simulink library "PacketizedNetworkLib"  (R2025b)
settings: Solver=VariableStepAuto  StartTime=0.0  StopTime=10.0  RelTol=1e-3
values from neighbouring files (symbols this model uses):
  dfeRef = [0.707106781187 -0.707106781187 0.707106781187 0.707106781187 -0.707106781187 0.707106781187 0.707106781187 0.707106781187 0.707106781187 0.707106781187 -0.707106781187 0.707106781187 ... (500 elements, 500x1)]    [networkParams.mat]
  L3payload = [0 0 0 1 0 0 0 0 1 1 1 0 ... (1040 elements, 1040x1)]    [networkParams.mat]
  ppdu_bb = [0 0 1 1 0 0 0 0 1 1 0 0 ... (2280 elements, 2280x1)]    [networkParams.mat]
  Ts = 1e-07    [networkParams.mat]
undefined symbols (not defined in the file or in its folder): AckDestAddre, DestAddre, dfilt, High, lambda, NodeAddre, pseed
libraries: $bdroot x19, hdlsllib x5, dspsigops x5, dspswit3 x3, simulink x3, dspindex x3, commdigbbndpm3 x2, simulink_extras x2, commfilt2 x2, commchan3 x1, dspmathops x1, dsparch4 x1
(part 3 of 3)

== stateflow chart PacketizedNetworkLib/PHY//MAC Transceiver/Subsystem/CSMA//CA MAC Layer ==
  note: Note:  802.11-like MAC with basic functions for DCF scenarios. PCF, HCF, MCF not implementaed.  For DCF, RTS and CTS  not implemented.
      |
      | 	    The MAC time unit is 8 times the symbol time (Ts), or 16 times the bit time.
      |           TxLength: data packet bit length divided by 16 = 529*(8000+464)/16.
      |   	    SLOT: backoff duration = TxLength/2.  With carrier sense or NAV, SLOT can be much smaller.
      |           CW: contention window length (number of SLOTs).
      | 	    BOTime: random back off time = randi([0 CW],1)*SLOT;
      |           AckLength: ack duration in MAC time units (number of ACK bits / 16)
      |           AckWaitTime: timer for AckWait state
      |           Retry is the retry number of a frame.
      |
      |           IFS Interfame space
      |           SigD Signal detection signal (i.e., carrier-sensing result)
      |           TxLength is an input from Link layer to indicate the bit length of the data packet.
      |           AckOK is the status of ACK packet CRC OK.
      |           TxDataTP is the time pading for the node to meet the SIFS time.
      |           TxAckTP is the time pading for the node to meet the SIFS time.
      |           TxDataDone is an output to LLC layer to show the current frame is transmitted OK.
      |           TxDataFail is an output to LLC layer to indicate that the current packet is failed.
  state Tx1 DATA and wait for ACK [group]
    state Reset
    state Reset1
    state TxOn
      en:
      TxTime=TxTime-1;
      TxDataOn=1;
    state AckWait
      en:
      AckWaitTime=AckWaitTime-1;
    state TurnOnTxSw
      en:
      TxDataTP=TxDataTP-1;
    Reset -> (junction 461) : {TxDataFail=0;}
    (junction 461) -> (junction 374)
    (junction 330) -> (junction 461) [order 1] : [Retry<SSCR]
        | {Retry=Retry+1;}
    (junction 327) -> (junction 374) [order 2] : {TxDataDone=0;}
    (junction 330) -> Reset [order 2] : [Retry==SSCR]
        | {TxDataFail=1;
        | Retry=0;
        | CW=CWmin; }
    Reset1 -> (junction 327)
    AckWait -> Reset1 [order 1] : [AckOk==1&&AckWaitTime>0]
        | {TxDataDone=1;
        | Retry=0;
        | CW=CWmin;}
    (junction 327) -> TurnOnTxSw [order 1] : [TxEn==1]
        | {BONum=0;
        | TxDataDone=0;
        | TxTime=TxLength;
        | TxDataTP=TP;}
    TxOn -> TxOn [order 2] : [TxTime>0]
    AckWait -> (junction 330) [order 2] : [AckWaitTime==0]
    TxOn -> AckWait [order 1] : [TxTime==0]
        | {AckWaitTime=AckLength+SIFS+20;
        | TxDataOn=0;}
    TurnOnTxSw -> TxOn [order 1] : [TxDataTP<=0]
    AckWait -> AckWait [order 3] : [AckWaitTime>0]
    TurnOnTxSw -> TurnOnTxSw [order 2]
  state Contention Window and Back Off [group]
    state IFS_Time
    state Backoff
      en:
      BOTime=BOTime-1;
    Backoff -> (junction 486) [order 1] : [SigD==1]
    IFS_Time -> IFS_Time [order 3] : [SigD==0]
        | {IFS=IFS-1;
        | SigSt=1;}
    IFS_Time -> (junction 473) [order 1] : [IFS==0]
    (junction 473) -> (junction 484) [order 2]
    (junction 484) -> (junction 354) [order 2]
    (junction 354) -> (junction 482) [order 2]
    (junction 473) -> Backoff [order 1] : [BOTime>0]
    (junction 484) -> Backoff [order 1] : [CW==CWmax]
        | {BOTime=randi([0 CW],1)*SLOT;}
    (junction 354) -> Backoff [order 1] : [Retry==0]
        | {BOTime=randi([0 CW],1)*SLOT;}
    (junction 482) -> Backoff : [CW<CWmax]
        | {CW=CW*2+1;
        | BOTime=randi([0 CW],1)*SLOT; }
    IFS_Time -> IFS_Time [order 5] : [RxErr==1]
        | {IFS=EIFS;}
    Backoff -> Backoff [order 3] : [BOTime>0&&SigD==0]
  state Tx ACK [group]
    state StandBy
    state RxDataOK
      en:
      TxAckTP=TxAckTP-1;
    state AckOn
      en:
      TxAckTime=TxAckTime-1;
      TxAckOn=1;
    (junction 434) -> StandBy [order 2]
    AckOn -> (junction 434) [order 1] : [TxAckTime==0]
        | {TxAckOn=0;
        | TxK=2;}
    StandBy -> (junction 394) [order 1] : [RxDataOk==1]
    (junction 394) -> RxDataOK : {TxAckTP=TP;}
    RxDataOK -> AckOn [order 1] : [TxAckTP<=0]
        | {TxAckTime=AckLength;}
    RxDataOK -> RxDataOK [order 2]
    AckOn -> AckOn [order 2]
  (default) -> (junction 372) : {
      | % Symbol time Ts = 1e-7, Bit time = Ts/2 = 0.5e-7.  MAC Clock Time is 16*(Ts/2) = 0.8 us
      | AckLength=400/16;      %Ack length = 400 bits, here "16" is the number of bits for MAC step size in bits
      | SLOT= 25;    %SLOT Time 20 us, 25*16*(Ts/2)= 20 us
      | DIFS = 62;    %DIFS Time  50 us, 62*16*(Ts/2)= 49.6 us
      | SIFS = 12;    %SIFS Time  10 us, 12*16*(Ts/2)= 9.6 us
      | EIFS = 100;  %EIFS Time  Ack Length + SIFS + DIFS, 20us + 50us + 10us = 80 us, 100*16*(Ts/2) = 80 us
      | TP=2;            % Tx/Rx Turnaround Time Padding for the node to meet SIFS time
      | rng(pseed) ;  % Rand Seed
      | CWmax=31;
      | CWmin=7;
      | TxDataFail=0;
      | TxDataDone=0;
      | BONum=0;
      | SSCR=10;
      | Retry=0;
      | %SigD=0;       % Signal detection is set to zero for the case that the carrier sense is not used in ALOHA MAC
      | }
  (junction 466) -> (junction 372) [order 2]
  (junction 374) -> (junction 466)
  (junction 372) -> StandBy : {CW=CWmin;
      | BONum=0;
      | BOTime=0;}
  (junction 466) -> (junction 488) [order 1] : [TxEn==1]
  (junction 486) -> (junction 488)
  (junction 488) -> (junction 452)
  (junction 434) -> (junction 452) [order 1] : [BOTime>0]
  StandBy -> (junction 452) [order 2] : [TxEn==1]
  (junction 452) -> IFS_Time : {IFS=DIFS;
      | SigSt=0;}
  IFS_Time -> (junction 452) [order 4] : [SigD==1&&SigSt==1]
  IFS_Time -> (junction 394) [order 2] : [RxDataOk==1]
  Backoff -> (junction 394) [order 2] : [RxDataOk==1]
  Backoff -> TurnOnTxSw [order 4] : [BOTime<=0]
      | {TxTime=TxLength;
      | TxDataTP=TP;}
  data: TxLength input double; TxEn input; RxDataOk input; AckOk input; TxDataFail output double; TxDataDone output double; AckLength local double; BONum local double; SIFS local double; CWmax local double; CW local double; SLOT local double; TxTime local double; TxDataOn output double; TxK local; TxAckOn output; BOTime output double; AckWaitTime output double; TxAckTP local; TxDataTP local; TP local; DIFS local; EIFS local; TxAckTime local; SigD input; SigSt local; RxErr input; IFS local; SSCR local; CWmin local; pseed parameter; Retry output

== matlab function PacketizedNetworkLib/PHY//MAC Transceiver/MATLAB Function ==
  data: ack output; NodeAddre parameter; DestAddre parameter; ppdu_bb parameter; AckDestAddre parameter
function ack = ackGenerator(NodeAddre, DestAddre, ppdu_bb, AckDestAddre)

%   Copyright 2017 The MathWorks, Inc.

persistent agc sync ackLength headCRC crcGenPHY crcGenMAC type version ...
            reserved sequenceNo fromAddress toAddress ackBits ackCRC 

% PHY Header

if isempty(crcGenMAC)
  agc  = ppdu_bb(1:50,1); %Load AGC signal
  sync = ppdu_bb(51:304); %Load Sync Signal
  ackLength = de2bi(64, 16, 'left-msb')';
  
  crcGenPHY = comm.CRCGenerator();
  temp = crcGenPHY(ackLength);
  headCRC = temp(17:32);
    
  % MAC header
  crcGenMAC = comm.CRCGenerator('z^32+z^26+z^23+z^22+z^16+z^12+z^11+z^10+z^8+z^7+z^5+z^4+z^2+z^1+1');
  type = [1 1 0 0]'; % [0 0 1 1] For Data Frame, [ 1 1 0 0] For ACK frame
  version = [0 0]';
  reserved = [0 0]';
  sequenceNo = [ 0 0 0 0 0 0 0 0 ]';
  
  toAddress = AckDestAddre';
  fromAddress = NodeAddre';

  ackBits=[type; ...
           version; ...
           reserved; ...
           toAddress; ...
           fromAddress; ...
           sequenceNo];

  ackCRC = crcGenMAC(ackBits);
end

ack =  [agc; ...
        sync; ...
        ackLength; ...
        headCRC; ...
        ackBits; ...
        ackCRC(end-31:end)];

== matlab function PacketizedNetworkLib/PHY//MAC Transceiver/MATLAB Function1 ==
  data: L3payload input size=1040; dataFrame output size=1472; NodeAddre parameter; DestAddre parameter; ppdu_bb parameter
function dataFrame = dataFrameGenerator(L3payload, NodeAddre, DestAddre, ppdu_bb)

%   Copyright 2017 The MathWorks, Inc.

persistent agc sync dataLength headCRC crcGenPHY crcGenMAC type version ...
            reserved sequenceNo fromAddress toAddress dataBits dataCRC ...
            time payload
          

% PHY Header

if isempty(crcGenMAC)
  agc  = ppdu_bb(1:50,1); %Load AGC signal
  sync = ppdu_bb(51:304); %Load Sync Signal
  dataLength = de2bi(64+length(L3payload)+32, 16, 'left-msb')';
  
  crcGenPHY = comm.CRCGenerator();
  temp = crcGenPHY(dataLength);
  headCRC = temp(17:32);
    
  % MAC header
  crcGenMAC = comm.CRCGenerator('z^32+z^26+z^23+z^22+z^16+z^12+z^11+z^10+z^8+z^7+z^5+z^4+z^2+z^1+1');
  type = [0 0 1 1]'; % [0 0 1 1] For Data Frame, [ 1 1 0 0] For ACK frame
  version = [0 0]';
  reserved = [0 0]';
  sequenceNo = [ 0 0 0 0 0 0 0 0 ]';
  time = zeros(32,1);
  
  fromAddress = NodeAddre';
  toAddress = DestAddre';

  payload = L3payload;
  
  dataBits=[type; ...
           version; ...
           reserved; ...
           toAddress; ...
           fromAddress; ...
           sequenceNo; ...
           time; ...
           payload];

  dataCRC = crcGenMAC(dataBits);
end

dataFrame =  [agc; ...
              sync; ...
              dataLength; ...
              headCRC; ...
              dataBits; ...
              dataCRC(end-31:end)];

== stateflow chart PacketizedNetworkLib/Logical Link Control/Logical Link Control ==
  state TxBackOn
    en:
    TxWaitTime=TxWaitTime-1;
    TxEn=0;
  state TxFailCount
    en:
    TxFlCnt=TxFlCnt+1 ;
  state TxPacket
    en:
    TxEn=1;
  note: Notes:
      |             TxWaitTime is the packet inter-arrival time. It represents multiples of 8*Ts.
      |             TxMore is a random number in [1 4], indicating additional segments transmissions.
      |             TxDataDone is an input from the MAC layer indicating that the current frame completed transmission.
      |             TxDataFail is an input from the MAC layer indicating that the current packet failed transmission.
      | 		TxDataBitsLength is the bit length of the data payload from layer #3 (network).
      |             TxLength is the frame length in multiples of 16 bits.
      |             StopSim is an output of the LLC that stops simulation when a frame completely fails transmission.
  (default) -> (junction 5) : {TxDataBitsLength=1040;  % M (Link payload)
      | TxFlCntMax=100;
      | TxLength=(TxDataBitsLength+464)/16; % 464 is the bit # of AGC+Header+MAC_Header+FCS
      | rng(pseed) ; % Poisson Rand Seed
      | TxFlCnt=0;
      | }
  TxFailCount -> (junction 5) [order 2] : [TxFlCnt<TxFlCntMax]
  TxFailCount -> (junction 10) [order 1] : [TxFlCnt==TxFlCntMax]
      | {StopSim=1;
      | TxEn=0;}
  (junction 5) -> TxBackOn : {
      | TxWaitTime=TxWaitUnits;
      | TxMore=randi([1 4], 1)-1;
      |  }
  TxPacket -> (junction 5) [order 1] : [TxDataDone==1&&TxMore<=0]
  TxBackOn -> TxBackOn [order 2]
  TxPacket -> TxFailCount [order 2] : [TxDataFail==1]
      | {TxEn=0;}
  TxBackOn -> TxPacket [order 1] : [TxWaitTime<=0]
  TxPacket -> TxPacket [order 3] : [TxDataDone==1]
      | {TxMore=TxMore-1;}
  data: TxDataDone input; TxDataFail input; StopSim output; TxEn output; TxDataBitsLength local; TxFlCnt local; TxFlCntMax local double; TxLength output; TxWaitTime output; TxMore output; pseed parameter; TxWaitUnits input

== matlab function PacketizedNetworkLib/Receiver/DFE /Sign_C  ==
  data: u input; y output
function y = fcn(u)
y=0.707*complex(sign(real(u)), sign(imag(u)));

== stateflow chart PacketizedNetworkLib/ALOHA MAC Layer ==
  state Delay
  state Reset
  state Tx1 DATA [group]
    state Reset1
    state AckWait
      en:
      AckWaitTime=AckWaitTime-1;
    state TxOn
      en:
      TxTime=TxTime-1;
      TxDataOn=1;
    state Delay2
      en:
      TxK=TxK-1;
    state TurnOnTxSw
      en:
      TxDataSIFS=TxDataSIFS-1;
      TxSwOn=1;
    state Backoff
      en:
      BOTime=BOTime-1;
    Reset1 -> (junction 327)
    (junction 327) -> TurnOnTxSw [order 1] : [TxEn==1]
        | {CW=15;
        | BONum=0;
        | TxDataDone=0;
        | TxTime=TxLength;
        | TxDataSIFS=SIFS;}
    AckWait -> Reset1 [order 1] : [AckOk==1&&AckWaitTime>0]
        | {TxDataDone=1;}
    TurnOnTxSw -> TxOn [order 1] : [TxDataSIFS<=0]
    TxOn -> Delay2 [order 1] : [TxTime==0]
        | {AckWaitTime=AckLength+64;
        | TxDataOn=0;
        | TxK=2;}
    Delay2 -> AckWait [order 1] : [TxK==0]
        | {TxSwOn=0;}
    Delay2 -> Delay2 [order 2]
    TurnOnTxSw -> TurnOnTxSw [order 2]
    Backoff -> TurnOnTxSw [order 3] : [BOTime<=0]
        | {BONum=BONum+1;
        | TxTime=TxLength;}
    TxOn -> TxOn [order 2] : [TxTime>0]
    AckWait -> AckWait [order 3] : [AckWaitTime>0]
    (junction 354) -> Backoff [order 1] : [BONum==0]
        | {BOTime=randi([0 CW],1)*SLOT;}
    (junction 354) -> Backoff [order 2] : {CW=CW*2+1;
        |  BOTime=randi([0 CW],1)*SLOT;}
    Backoff -> Backoff [order 2] : [BOTime>0]
  state StandBy
  state Tx ACK [group]
    state Delay1
      en:
      TxK=TxK-1;
    state RxDataOK
      en:
      TxAckSIFS=TxAckSIFS-1;
      TxSwOn=1;
    state AckOn
      en:
      TxAckTime=TxAckTime-1;
      TxAckOn=1;
      TxSwOn=1;
    (junction 394) -> RxDataOK : {TxAckSIFS=SIFS;}
    Delay1 -> Delay1 [order 2]
    AckOn -> Delay1 [order 1] : [TxAckTime==0]
        | {TxAckOn=0;
        | TxK=2;}
    RxDataOK -> AckOn [order 1] : [TxAckSIFS<=0]
        | {TxAckTime=AckLength;}
    RxDataOK -> RxDataOK [order 2]
    AckOn -> AckOn [order 2]
  note: Note: The MAC time unit is 8 times the symbol time (Ts), or 16 times the bit time.
      |           TxLength: data packet bit length divided by 16 = 529*(8000+464)/16.
      |   	    SLOT: backoff duration = TxLength/2.  With carrier sense or NAV, SLOT can be much smaller.
      |              In 802.11, SLOT is 20 us (5us turn around and 15us energy detection)
      |           CW: contention window length (number of SLOTs).
      | 	    BOTime: random back off time = randi([0 CW],1)*SLOT;
      |           SIFS: short interframe spacing is the idle time between the end of a data packet and the start of the ACK packet. It is set to 2 MAC time units (= 2x16 bits).
      |           AckLength: ack duration in MAC time units (number of ACK bits / 16)
      |           AckWaitTime: timer for AckWait state
      |           BoNum: number of backoff attempts.
      |
      |           AckOK: status of ACK packet CRC.
      |
      |           TxDataDone: output to LLC sublayer indicating that the current packet is transmitted OK.
      |           TxDataFail: output to LLC sublayer indicating that the current packet has failed.
  (default) -> (junction 372) : {
      | SLOT=floor(TxLength/2);     %SLOT time
      | SIFS=2;                        % Tx/Rx Turnaround
      | AckLength=400/16;      %Ack length = 400 bits, here "16" is the number of bits for MAC step size in bits
      | CWmax=31;
      | rng(pseed);
      | TxDataFail=0;
      | TxDataDone=0;
      | BONum=0;
      | SigD=0;       % Signal detection is set to zero for the case that the carrier sense is not used
      | }
  (junction 374) -> Delay
  Reset -> (junction 374) : {TxDataFail=0;}
  Delay -> (junction 372)
  (junction 327) -> (junction 374) [order 2] : {TxDataDone=0;}
  (junction 372) -> StandBy : {CW=15;
      | BONum=0;
      | BOTime=0;}
  (junction 330) -> Reset [order 2] : [CW==CWmax]
      | {TxDataFail=1;}
  AckWait -> (junction 330) [order 2] : [AckWaitTime==0]
  StandBy -> TurnOnTxSw [order 2] : [TxEn==1&&SigD==0]
      | {TxTime=TxLength;
      | TxDataSIFS=SIFS;}
  (junction 330) -> (junction 354) [order 1] : [CW<CWmax]
  (junction 434) -> StandBy [order 2]
  (junction 434) -> Backoff [order 1] : [BOTime>0]
  Delay1 -> (junction 434) [order 1] : [TxK==0]
      | {TxSwOn=0;}
  StandBy -> (junction 394) [order 1] : [RxDataOk==1]
  Backoff -> (junction 394) [order 1] : [RxDataOk==1]
  data: TxLength input double; TxEn input; RxDataOk input; AckOk input; TxDataFail output double; TxDataDone output double; AckLength local double; BONum local double; SIFS local double; CWmax local double; CW local double; SLOT local double; TxTime local double; TxDataOn output double; SigD local; TxK local; TxAckOn output; BOTime output double; AckWaitTime output double; TxAckTime local; TxDataSIFS local; TxAckSIFS local; TxSwOn local; pseed parameter

== stateflow chart PacketizedNetworkLib/CSMA//CA MAC Layer ==
  note: Note:  802.11-like MAC with basic functions for DCF scenarios. PCF, HCF, MCF not implementaed.  For DCF, RTS and CTS  not implemented.
      |
      | 	    The MAC time unit is 8 times the symbol time (Ts), or 16 times the bit time.
      |           TxLength: data packet bit length divided by 16 = 529*(8000+464)/16.
      |   	    SLOT: backoff duration = TxLength/2.  With carrier sense or NAV, SLOT can be much smaller.
      |           CW: contention window length (number of SLOTs).
      | 	    BOTime: random back off time = randi([0 CW],1)*SLOT;
      |           AckLength: ack duration in MAC time units (number of ACK bits / 16)
      |           AckWaitTime: timer for AckWait state
      |           Retry is the retry number of a frame.
      |
      |           IFS Interfame space
      |           SigD Signal detection signal (i.e., carrier-sensing result)
      |           TxLength is an input from Link layer to indicate the bit length of the data packet.
      |           AckOK is the status of ACK packet CRC OK.
      |           TxDataTP is the time pading for the node to meet the SIFS time.
      |           TxAckTP is the time pading for the node to meet the SIFS time.
      |           TxDataDone is an output to LLC layer to show the current frame is transmitted OK.
      |           TxDataFail is an output to LLC layer to indicate that the current packet is failed.
  state Tx1 DATA and wait for ACK [group]
    state Reset
    state Reset1
    state TxOn
      en:
      TxTime=TxTime-1;
      TxDataOn=1;
    state AckWait
      en:
      AckWaitTime=AckWaitTime-1;
    state TurnOnTxSw
      en:
      TxDataTP=TxDataTP-1;
    Reset -> (junction 461) : {TxDataFail=0;}
    (junction 461) -> (junction 374)
    (junction 330) -> (junction 461) [order 1] : [Retry<SSCR]
        | {Retry=Retry+1;}
    (junction 327) -> (junction 374) [order 2] : {TxDataDone=0;}
    (junction 330) -> Reset [order 2] : [Retry==SSCR]
        | {TxDataFail=1;
        | Retry=0;
        | CW=CWmin; }
    Reset1 -> (junction 327)
    AckWait -> Reset1 [order 1] : [AckOk==1&&AckWaitTime>0]
        | {TxDataDone=1;
        | Retry=0;
        | CW=CWmin;}
    (junction 327) -> TurnOnTxSw [order 1] : [TxEn==1]
        | {BONum=0;
        | TxDataDone=0;
        | TxTime=TxLength;
        | TxDataTP=TP;}
    TxOn -> TxOn [order 2] : [TxTime>0]
    AckWait -> (junction 330) [order 2] : [AckWaitTime==0]
    TxOn -> AckWait [order 1] : [TxTime==0]
        | {AckWaitTime=AckLength+SIFS+20;
        | TxDataOn=0;}
    TurnOnTxSw -> TxOn [order 1] : [TxDataTP<=0]
    AckWait -> AckWait [order 3] : [AckWaitTime>0]
    TurnOnTxSw -> TurnOnTxSw [order 2]
  state Contention Window and Back Off [group]
    state IFS_Time
    state Backoff
      en:
      BOTime=BOTime-1;
    Backoff -> (junction 486) [order 1] : [SigD==1]
    IFS_Time -> IFS_Time [order 3] : [SigD==0]
        | {IFS=IFS-1;
        | SigSt=1;}
    IFS_Time -> (junction 473) [order 1] : [IFS==0]
    (junction 473) -> (junction 484) [order 2]
    (junction 484) -> (junction 354) [order 2]
    (junction 354) -> (junction 482) [order 2]
    (junction 473) -> Backoff [order 1] : [BOTime>0]
    (junction 484) -> Backoff [order 1] : [CW==CWmax]
        | {BOTime=randi([0 CW],1)*SLOT;}
    (junction 354) -> Backoff [order 1] : [Retry==0]
        | {BOTime=randi([0 CW],1)*SLOT;}
    (junction 482) -> Backoff : [CW<CWmax]
        | {CW=CW*2+1;
        | BOTime=randi([0 CW],1)*SLOT; }
    IFS_Time -> IFS_Time [order 5] : [RxErr==1]
        | {IFS=EIFS;}
    Backoff -> Backoff [order 3] : [BOTime>0&&SigD==0]
  state Tx ACK [group]
    state StandBy
    state RxDataOK
      en:
      TxAckTP=TxAckTP-1;
    state AckOn
      en:
      TxAckTime=TxAckTime-1;
      TxAckOn=1;
    (junction 434) -> StandBy [order 2]
    AckOn -> (junction 434) [order 1] : [TxAckTime==0]
        | {TxAckOn=0;
        | TxK=2;}
    StandBy -> (junction 394) [order 1] : [RxDataOk==1]
    (junction 394) -> RxDataOK : {TxAckTP=TP;}
    RxDataOK -> AckOn [order 1] : [TxAckTP<=0]
        | {TxAckTime=AckLength;}
    RxDataOK -> RxDataOK [order 2]
    AckOn -> AckOn [order 2]
  (default) -> (junction 372) : {
      | % Symbol time Ts = 1e-7, Bit time = Ts/2 = 0.5e-7.  MAC Clock Time is 16*(Ts/2) = 0.8 us
      | AckLength=400/16;      %Ack length = 400 bits, here "16" is the number of bits for MAC step size in bits
      | SLOT= 25;    %SLOT Time 20 us, 25*16*(Ts/2)= 20 us
      | DIFS = 62;    %DIFS Time  50 us, 62*16*(Ts/2)= 49.6 us
      | SIFS = 12;    %SIFS Time  10 us, 12*16*(Ts/2)= 9.6 us
      | EIFS = 100;  %EIFS Time  Ack Length + SIFS + DIFS, 20us + 50us + 10us = 80 us, 100*16*(Ts/2) = 80 us
      | TP=2;            % Tx/Rx Turnaround Time Padding for the node to meet SIFS time
      | rng(pseed) ;  % Rand Seed
      | CWmax=31;
      | CWmin=7;
      | TxDataFail=0;
      | TxDataDone=0;
      | BONum=0;
      | SSCR=10;
      | Retry=0;
      | %SigD=0;       % Signal detection is set to zero for the case that the carrier sense is not used in ALOHA MAC
      | }
  (junction 466) -> (junction 372) [order 2]
  (junction 374) -> (junction 466)
  (junction 372) -> StandBy : {CW=CWmin;
      | BONum=0;
      | BOTime=0;}
  (junction 466) -> (junction 488) [order 1] : [TxEn==1]
  (junction 486) -> (junction 488)
  (junction 488) -> (junction 452)
  (junction 434) -> (junction 452) [order 1] : [BOTime>0]
  StandBy -> (junction 452) [order 2] : [TxEn==1]
  (junction 452) -> IFS_Time : {IFS=DIFS;
      | SigSt=0;}
  IFS_Time -> (junction 452) [order 4] : [SigD==1&&SigSt==1]
  IFS_Time -> (junction 394) [order 2] : [RxDataOk==1]
  Backoff -> (junction 394) [order 2] : [RxDataOk==1]
  Backoff -> TurnOnTxSw [order 4] : [BOTime<=0]
      | {TxTime=TxLength;
      | TxDataTP=TP;}
  data: TxLength input double; TxEn input; RxDataOk input; AckOk input; TxDataFail output double; TxDataDone output double; AckLength local double; BONum local double; SIFS local double; CWmax local double; CW local double; SLOT local double; TxTime local double; TxDataOn output double; TxK local; TxAckOn output; BOTime output double; AckWaitTime output double; TxAckTP local; TxDataTP local; TP local; DIFS local; EIFS local; TxAckTime local; SigD input; SigSt local; RxErr input; IFS local; SSCR local; CWmin local; pseed parameter; Retry output
